simulink model "HaulageOptimizedOperationSimulation"  (R2026a)
settings: Solver=FixedStepDiscrete  StopTime=1400  FixedStep=1
libraries: simulink x18
(part 2 of 2)

== matlab function HaulageOptimizedOperationSimulation/Baseline Operation Pipeline/Longitudinal Motion Equations ==
  data: safeSpeed_kph input size=1; speed_kph output size=1; routeVector input size=7; trackingTau_s input size=1; totalRouteDistance input; cumDistance_m output size=1; stepDistance_m output size=1; stepTime_s output size=1
function [speed_kph, cumDistance_m, stepDistance_m, stepTime_s] = f(safeSpeed_kph, routeVector, trackingTau_s, totalRouteDistance)
%#codegen
dt = 1;
persistent speed_mps distance_m
if isempty(speed_mps)
    speed_mps = 0.0;
    distance_m = 0.0;
end
payload_t = routeVector(5);
routeDone = routeVector(7);
speed_kph = speed_mps * 3.6;
cumDistance_m = distance_m;
stepDistance_m = 0.0;
stepTime_s = 0.0;
if routeDone < 0.5
    target_mps = safeSpeed_kph / 3.6;
    if payload_t <= 1.0
        maxAccel = 0.55;
        maxDecel = 0.75;
    elseif payload_t < 225.0
        maxAccel = 0.42;
        maxDecel = 0.68;
    else
        maxAccel = 0.35;
        maxDecel = 0.62;
    end
    speedError = target_mps - speed_mps;
    desiredAccel = speedError / max(trackingTau_s, dt);
    accel = min(max(desiredAccel, -maxDecel), maxAccel);
    speed_mps = max(speed_mps + accel * dt, 0.1);
    remaining_m = max(totalRouteDistance - distance_m, 0.0);
    stepDistance_m = min(speed_mps * dt, remaining_m);
    stepTime_s = stepDistance_m / max(speed_mps, 0.1);
    distance_m = distance_m + stepDistance_m;
end
speed_kph = speed_mps * 3.6;
cumDistance_m = distance_m;

== matlab function HaulageOptimizedOperationSimulation/Optimized Operation Pipeline/Energy SFC Equations ==
  data: speed_kph input size=1; cumFuel_l output size=1; stepDistance_m input size=1; stepTime_s input size=1; routeVector input size=7; vehicleParams input size=6; fuelRate_lph output size=1; instSfc_l_per_tkm output size=1; productiveTonKm output size=1
function [cumFuel_l, fuelRate_lph, instSfc_l_per_tkm, productiveTonKm] = f(speed_kph, stepDistance_m, stepTime_s, routeVector, vehicleParams)
%#codegen
emptyMass = vehicleParams(1);
idleFuelRate = vehicleParams(2);
maxFuelRate = vehicleParams(3);
frontalArea = vehicleParams(4);
dragCoefficient = vehicleParams(5);
drivetrainEfficiency = vehicleParams(6);
persistent fuel_l prod_tkm
if isempty(fuel_l)
    fuel_l = 0.0;
    prod_tkm = 0.0;
end
effGrade_pct = routeVector(2);
payload_t = routeVector(5);
routeDone = routeVector(7);
fuelRate_lph = idleFuelRate;
instSfc_l_per_tkm = NaN;
cumFuel_l = fuel_l;
productiveTonKm = prod_tkm;
if routeDone < 0.5 && stepTime_s > 0.0
    speed_mps = speed_kph / 3.6;
    g = 9.81;
    rho = 1.225;
    dieselEnergy_kWhPerL = 9.7;
    mass_kg = emptyMass + payload_t * 1000.0;
    gradeForce_N = mass_kg * g * (effGrade_pct / 100.0);
    aeroForce_N = 0.5 * rho * dragCoefficient * frontalArea * speed_mps^2;
    tractiveForce_N = gradeForce_N + aeroForce_N;
    if tractiveForce_N <= 0.0
        fuelRate_lph = idleFuelRate;
    else
        wheelPower_kW = tractiveForce_N * speed_mps / 1000.0;
        fuelRate_lph = idleFuelRate + wheelPower_kW / (drivetrainEfficiency * dieselEnergy_kWhPerL);
    end
    fuelRate_lph = min(max(fuelRate_lph, idleFuelRate), maxFuelRate);
    fuel_l = fuel_l + fuelRate_lph * stepTime_s / 3600.0;
    if payload_t > 0.0
        prod_tkm = prod_tkm + payload_t * stepDistance_m / 1000.0;
        instSfc_l_per_tkm = fuelRate_lph / max(payload_t * speed_kph, eps);
    end
end
cumFuel_l = fuel_l;
productiveTonKm = prod_tkm;

== matlab function HaulageOptimizedOperationSimulation/Optimized Operation Pipeline/Longitudinal Motion Equations ==
  data: safeSpeed_kph input size=1; speed_kph output size=1; routeVector input size=7; trackingTau_s input size=1; totalRouteDistance input; cumDistance_m output size=1; stepDistance_m output size=1; stepTime_s output size=1
function [speed_kph, cumDistance_m, stepDistance_m, stepTime_s] = f(safeSpeed_kph, routeVector, trackingTau_s, totalRouteDistance)
%#codegen
dt = 1;
persistent speed_mps distance_m
if isempty(speed_mps)
    speed_mps = 0.0;
    distance_m = 0.0;
end
payload_t = routeVector(5);
routeDone = routeVector(7);
speed_kph = speed_mps * 3.6;
cumDistance_m = distance_m;
stepDistance_m = 0.0;
stepTime_s = 0.0;
if routeDone < 0.5
    target_mps = safeSpeed_kph / 3.6;
    if payload_t <= 1.0
        maxAccel = 0.55;
        maxDecel = 0.75;
    elseif payload_t < 225.0
        maxAccel = 0.42;
        maxDecel = 0.68;
    else
        maxAccel = 0.35;
        maxDecel = 0.62;
    end
    speedError = target_mps - speed_mps;
    desiredAccel = speedError / max(trackingTau_s, dt);
    accel = min(max(desiredAccel, -maxDecel), maxAccel);
    speed_mps = max(speed_mps + accel * dt, 0.1);
    remaining_m = max(totalRouteDistance - distance_m, 0.0);
    stepDistance_m = min(speed_mps * dt, remaining_m);
    stepTime_s = stepDistance_m / max(speed_mps, 0.1);
    distance_m = distance_m + stepDistance_m;
end
speed_kph = speed_mps * 3.6;
cumDistance_m = distance_m;
